simulink library "bldc_plant_lib"  (R2023a)
settings: Solver=VariableStepAuto  StartTime=0.0  StopTime=10.0  RelTol=1e-3
values from neighbouring files (symbols this model uses):
  A = arrayfun(@(n) harmAmp(t, x, n*f1, t1, Tw), 1:nMax)    [bldc_kpi.m]    (also in bldc_ss_indicators.m = 2/numel(x)*abs(sum(x.*exp(-1j*2*pi*f*t))))
  P = bldc_set_encoder(P, 0, 0)    [bldc_params.m]
libraries: simulink x1, spsPermanentMagnetSynchronousMachineLib x1, spsUniversalBridgeLib x1, spsDCVoltageSourceLib x1
settings Model: Creator=PC  LastModifiedBy=PC

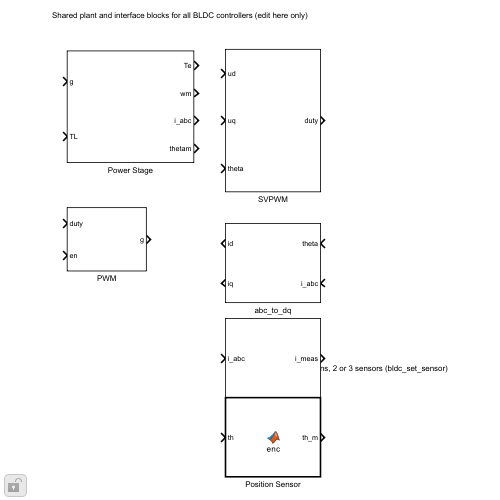
[thumbnail: Simulink's stored preview of the top-level diagram]
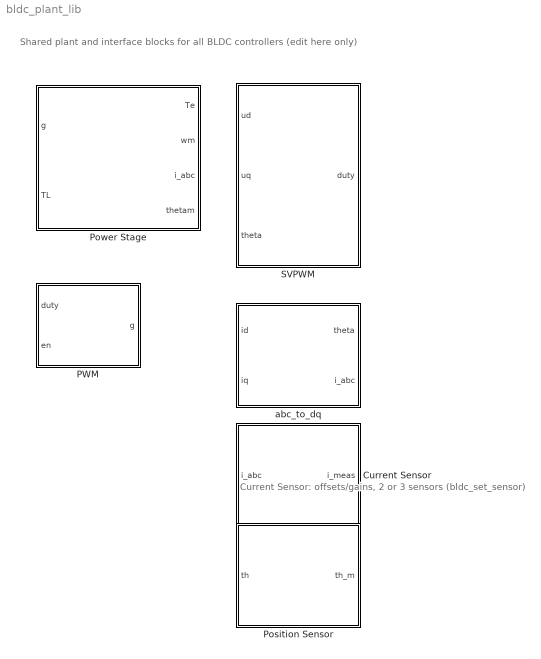
== system bldc_plant_lib ==
  note: Shared plant and interface blocks for all BLDC controllers (edit here only)
  note: Current Sensor: offsets/gains, 2 or 3 sensors (bldc_set_sensor)
  Current Sensor : Subsystem  Description=Phase-current sensors: i_meas = P.CS.M*(P.CS.gain.*i_abc + P.CS.off). Ideal by default (bldc_set_sensor).
  PWM : Subsystem
  Position Sensor : MATLAB Function  Description=Position sensor: quantized mechanical angle + mounting offset (P.ENC, bldc_set_encoder). Ideal by default.  TreatAsAtomicUnit=on
  Power Stage : Subsystem
  SVPWM : Subsystem
  abc_to_dq : Subsystem

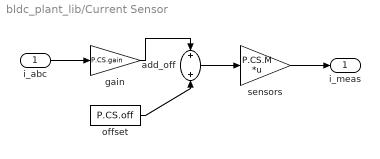
== system bldc_plant_lib/Current Sensor ==
  i_abc : Inport
  add_off : Sum
  gain : Gain  Gain=P.CS.gain
  offset : Constant  Value=P.CS.off
  sensors : Gain  Gain=P.CS.M  Multiplication=Matrix(K*u)
  i_meas : Outport
  wires:
  i_abc/1 -> gain/1
  gain/1 -> add_off/1
  offset/1 -> add_off/2
  add_off/1 -> sensors/1
  sensors/1 -> i_meas/1

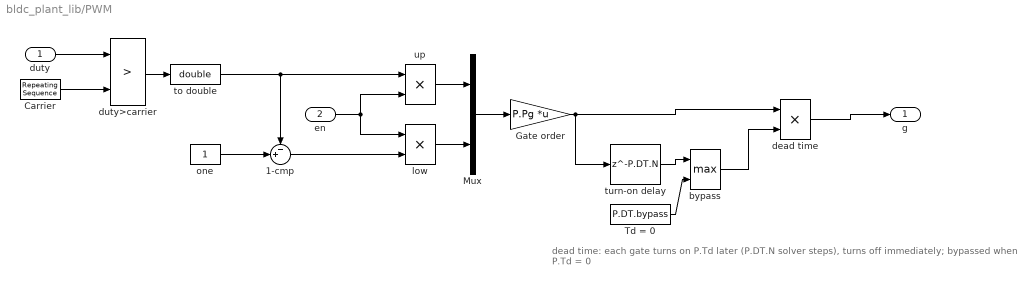
== system bldc_plant_lib/PWM ==
  note: dead time: each gate turns on P.Td later (P.DT.N solver steps), turns off immediately; bypassed when P.Td = 0
  duty : Inport
  en : Inport  Port=2
  1-cmp : Sum  Inputs=-+|
  Carrier : simulink/Sources/Repeating Sequence  rep_seq_t=[0 P.Ts/2 P.Ts]  rep_seq_y=[0 1 0]
  Gate order : Gain  Gain=P.Pg  Multiplication=Matrix(K*u)
  Mux : Mux  Inputs=2
  Td = 0 : Constant  Value=P.DT.bypass
  bypass : MinMax  Function=max  Inputs=2
  dead time : Product
  duty>carrier : RelationalOperator  Operator=>
  low : Product
  one : Constant
  to double : DataTypeConversion  OutDataTypeStr=double  SaturateOnIntegerOverflow=off  RndMeth=Floor
  turn-on delay : Delay  DelayLength=P.DT.N  InitialCondition=0  SampleTime=P.dt
  up : Product
  g : Outport
  wires:
  up/1 -> Mux/1
  to double/1 -> up/1, 1-cmp/1
  one/1 -> 1-cmp/2
  low/1 -> Mux/2
  en/1 -> low/1, up/2
  duty>carrier/1 -> to double/1
  duty/1 -> duty>carrier/1
  Mux/1 -> Gate order/1
  Carrier/1 -> duty>carrier/2
  1-cmp/1 -> low/2
  Gate order/1 -> dead time/1, turn-on delay/1
  turn-on delay/1 -> bypass/1
  Td = 0/1 -> bypass/2
  bypass/1 -> dead time/2
  dead time/1 -> g/1

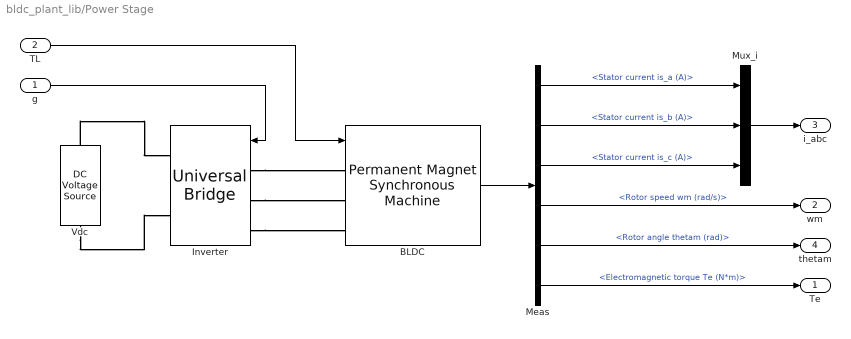
== system bldc_plant_lib/Power Stage ==
  g : Inport
  TL : Inport  Port=2
  BLDC : spsPermanentMagnetSynchronousMachineLib/Permanent Magnet Synchronous Machine  NbPhases=3  FluxDistribution=Trapezoidal  RotorType=Round  MechanicalLoad=Torque Tm  PresetModel=No  ShowDetailedParameters=on  MeasurementBus=off  Resistance=P.R*P.MIS.R  Inductance=P.L*P.MIS.L  dqInductances=[8.5e-3,8.5e-3]  La=0.000395  MachineConstant=Flux linkage established by magnets (V.s)  Flux=P.lam*P.MIS.lam  VoltageCst=286.5133  TorqueCst=2.736  Flat=P.MIS.flat  Mechanical=[P.J P.B P.p 0]  PolePairs=4  InitialConditions=[0 0 0 0]  InitialConditions5ph=[0 0 0 0 0 0]  RefAngle=90 degrees behind phase A axis (modified Park)  IterativeDiscreteModel=Trapezoidal non iterative  TsBlock=-1  TsPowergui=0
  Inverter : spsUniversalBridgeLib/Universal Bridge  Arms=3  SnubberResistance=1e5  SnubberCapacitance=inf  Device=IGBT / Diodes  Ron=1e-3  Lon=0  ForwardVoltages=P.Vf  ForwardVoltage=0  GTOparameters=[ 10e-6 , 20e-6 ]  IGBTparameters=[ 1e-6 , 2e-6 ]  Measurements=None  Measurements_2=None  converterType=Inverter
  Meas : BusSelector  OutputSignals=Stator current is_a (A),Stator current is_b (A),Stator current is_c (A),Rotor speed wm (rad/s),Rotor angle thetam (rad),Electromagnetic torque Te (N*m)
  Mux_i : Mux  Inputs=3
  Vdc : spsDCVoltageSourceLib/DC Voltage Source  Amplitude=P.Vdc  Measurements=None
  Te : Outport
  wm : Outport  Port=2
  i_abc : Outport  Port=3
  thetam : Outport  Port=4
  wires:
  g/1 -> Inverter/1
  TL/1 -> BLDC/1
  Mux_i/1 -> i_abc/1
  Meas/6 -> Te/1  "<Electromagnetic torque Te (N*m)>"
  Meas/5 -> thetam/1  "<Rotor angle thetam (rad)>"
  Meas/4 -> wm/1  "<Rotor speed wm (rad/s)>"
  Meas/3 -> Mux_i/3  "<Stator current is_c (A)>"
  Meas/2 -> Mux_i/2  "<Stator current is_b (A)>"
  Meas/1 -> Mux_i/1  "<Stator current is_a (A)>"
  BLDC/1 -> Meas/1
  connections:
  Vdc/RConn1 -- Inverter/RConn1
  Vdc/LConn1 -- Inverter/RConn2
  Inverter/LConn3 -- BLDC/LConn3
  Inverter/LConn2 -- BLDC/LConn2
  Inverter/LConn1 -- BLDC/LConn1

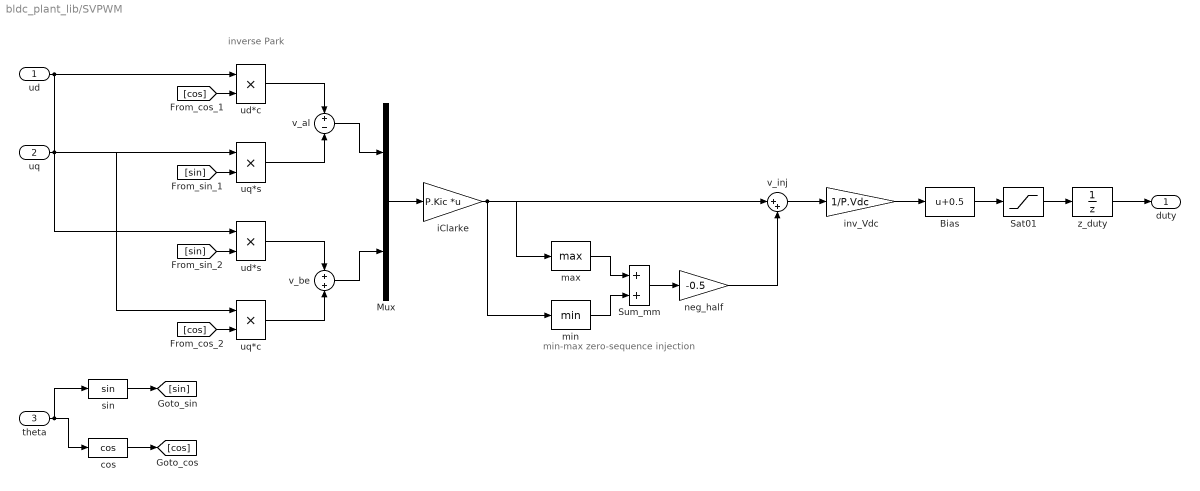
== system bldc_plant_lib/SVPWM ==
  note: min-max zero-sequence injection
  note: inverse Park
  ud : Inport
  uq : Inport  Port=2
  theta : Inport  Port=3
  Bias : Bias  Bias=0.5  SaturateOnIntegerOverflow=off
  Mux : Mux  Inputs=2
  Sat01 : Saturate  UpperLimit=1  LowerLimit=0
  Sum_mm : Sum
  cos : Trigonometry  Operator=cos
  iClarke : Gain  Gain=P.Kic  Multiplication=Matrix(K*u)
  inv_Vdc : Gain  Gain=1/P.Vdc
  max : MinMax  Function=max
  min : MinMax
  neg_half : Gain  Gain=-0.5
  sin : Trigonometry
  ud*c : Product
  ud*s : Product
  uq*c : Product
  uq*s : Product
  v_al : Sum  Inputs=+|-
  v_be : Sum  Inputs=+|+
  v_inj : Sum  Inputs=|++
  z_duty : UnitDelay  SampleTime=P.Ts  HasFrameUpgradeWarning=on
  duty : Outport
  wires:
  z_duty/1 -> duty/1
  v_inj/1 -> inv_Vdc/1
  v_be/1 -> Mux/2
  v_al/1 -> Mux/1
  uq*s/1 -> v_al/2
  uq*c/1 -> v_be/2
  uq/1 -> uq*s/1, uq*c/1
  ud*s/1 -> v_be/1
  ud*c/1 -> v_al/1
  ud/1 -> ud*s/1, ud*c/1
  theta/1 -> sin/1, cos/1
  neg_half/1 -> v_inj/2
  min/1 -> Sum_mm/2
  max/1 -> Sum_mm/1
  inv_Vdc/1 -> Bias/1
  iClarke/1 -> v_inj/1, min/1, max/1
  Sum_mm/1 -> neg_half/1
  Sat01/1 -> z_duty/1
  Mux/1 -> iClarke/1
  Bias/1 -> Sat01/1
  [cos] -> uq*c/2
  [cos] -> ud*c/2
  cos/1 -> [cos]
  [sin] -> ud*s/2
  [sin] -> uq*s/2
  sin/1 -> [sin]

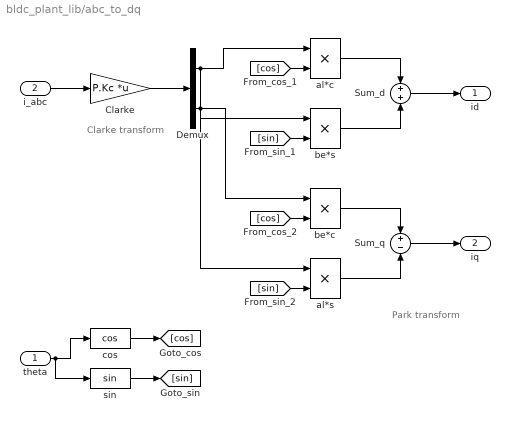
== system bldc_plant_lib/abc_to_dq ==
  note: Park transform
  note: Clarke transform
  theta : Inport
  i_abc : Inport  Port=2
  Clarke : Gain  Gain=P.Kc  Multiplication=Matrix(K*u)
  Demux : Demux  Outputs=2
  Sum_d : Sum  Inputs=+|+
  Sum_q : Sum  Inputs=+|-
  al*c : Product
  al*s : Product
  be*c : Product
  be*s : Product
  cos : Trigonometry  Operator=cos
  sin : Trigonometry
  id : Outport
  iq : Outport  Port=2
  wires:
  theta/1 -> sin/1, cos/1
  i_abc/1 -> Clarke/1
  be*s/1 -> Sum_d/2
  be*c/1 -> Sum_q/1
  al*s/1 -> Sum_q/2
  al*c/1 -> Sum_d/1
  Sum_q/1 -> iq/1
  Sum_d/1 -> id/1
  Demux/2 -> be*s/1, be*c/1
  Demux/1 -> al*s/1, al*c/1
  Clarke/1 -> Demux/1
  [sin] -> al*s/2
  [sin] -> be*s/2
  sin/1 -> [sin]
  [cos] -> be*c/2
  [cos] -> al*c/2
  cos/1 -> [cos]

== matlab function bldc_plant_lib/Position Sensor ==
  data: th input; th_m output; P parameter
function th_m = enc(th, P)
% position sensor: quantization + mounting offset (P.ENC, Common/bldc_set_encoder.m)
th_m = th;
if P.ENC.on
    th_m = P.ENC.q*floor(th/P.ENC.q);
end
if P.ENC.off ~= 0
    th_m = th_m + P.ENC.off;
end
